simulink model "basebot_turn"  (R2026a)
settings: Solver=VariableStepAuto  MaxStep=1e-4
values from neighbouring files (symbols this model uses):
  B = 0.15    [buildExercise1Models.m]    (also in driveModel.m; driveSquare.m; finalProjectModel.m; squareModel.m = 0.14)
  den = conv([L R], [J D]) + [0 0 K^2]    [compareRobot.m]    (also in driveModel.m; driveSquare.m; piDesign.mat = [3.18211752541e-08 2.39694947115e-05 7.04575028668e-05]; samplingModel.m)
  gear = 9.6    [buildExercise1Models.m]    (also in compareRobot.m; driveModel.m; driveSquare.m; finalProjectModel.m)
  Ki = Kp / 0.04    (= 0.5)    [driveSquare.m]
  Kit = Kpt / 0.15    (= 3.33333333333)    [driveSquare.m]
  Kp = runs{n,2}    [compareRobot.m]    (also in driveSquare.m = 0.02; piDesign.m = 0.13; piDesign.mat = 0.13; samplingModel.m = 0.05)
  Kph = 5    [driveSquare.m]    (also in squareModel.m = 1 / magH(idxWc))
  Kpt = 0.5    [driveSquare.m]
  maxTurn = 5    [driveSquare.m]
  num = K    [compareRobot.m]    (also in driveModel.m; driveSquare.m; piDesign.mat = 0.00812424172394; samplingModel.m)
  r = 0.0315    [compareRobot.m]    (also in driveModel.m; driveSquare.m; finalProjectModel.m; samplingModel.m)
  T = 0.010    (= 0.01)    [compareRobot.m]    (also in piDesign.mat; samplingModel.m; transferFunction.m)
  Ts = 0.001;'    [buildExercise1Models.m]    (also in compareRobot.m = round(median(diff(t)), 4); driveModel.m = 0.001; driveSquare.m = 0.001; finalProjectModel.m = 0.001)
  Vmax = 9    [compareRobot.m]    (also in driveModel.m; driveSquare.m; finalProjectModel.m; piDesign.m = 8)
libraries: slpidlib x3
settings Model: Creator=bidaze  LastModifiedBy=bidaze

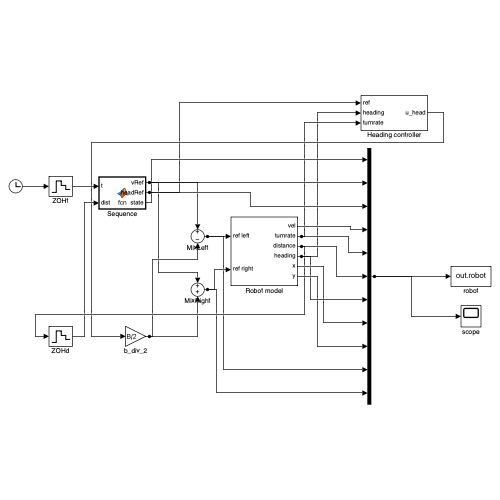
[thumbnail: Simulink's stored preview of the top-level diagram]
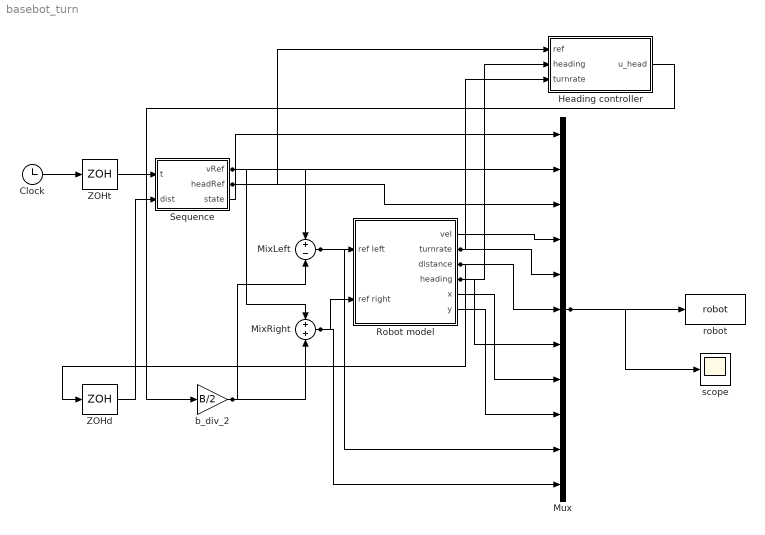
== system basebot_turn ==
  Clock : Clock
  Heading controller : Subsystem
  MixLeft : Sum  Inputs=+-
  MixRight : Sum
  Mux : Mux  Inputs=11
  Robot model : Subsystem
  Sequence : MATLAB Function  TreatAsAtomicUnit=on
  ZOHd : ZeroOrderHold  SampleTime=Ts
  ZOHt : ZeroOrderHold  SampleTime=Ts
  b_div_2 : Gain  Gain=B/2
  robot : ToWorkspace  VariableName=robot  SaveFormat=Timeseries  SampleTime=-1
  scope : Scope
  wires:
  Robot model/5(x) -> Mux/8
  Mux/1 -> scope/1, robot/1
  Robot model/3(distance) -> Mux/6, ZOHd/1
  Robot model/6(y) -> Mux/9
  ZOHt/1 -> Sequence/1(t)
  MixRight/1 -> Robot model/2(ref right), Mux/11
  ZOHd/1 -> Sequence/2(dist)
  Robot model/1(vel) -> Mux/4
  MixLeft/1 -> Robot model/1(ref left), Mux/10
  Robot model/4(heading) -> Mux/7, Heading controller/2(heading)
  Sequence/3(state) -> Mux/1
  Sequence/2(headRef) -> Heading controller/1(ref), Mux/3
  Heading controller/1(u_head) -> b_div_2/1
  Clock/1 -> ZOHt/1
  Robot model/2(turnrate) -> Mux/5, Heading controller/3(turnrate)
  b_div_2/1 -> MixLeft/2, MixRight/2
  Sequence/1(vRef) -> Mux/2, MixLeft/1, MixRight/1

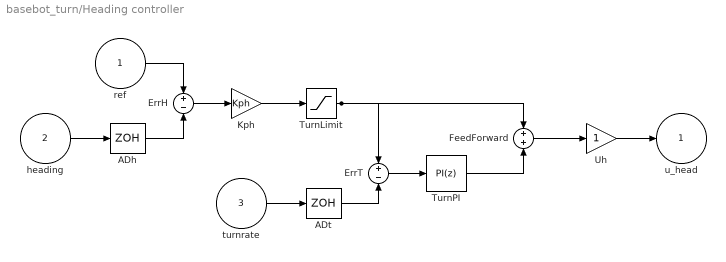
== system basebot_turn/Heading controller ==
  ref : Inport
  heading : Inport  Port=2
  turnrate : Inport  Port=3
  ADh : ZeroOrderHold  SampleTime=Ts
  ADt : ZeroOrderHold  SampleTime=Ts
  ErrH : Sum  Inputs=+-
  ErrT : Sum  Inputs=+-
  FeedForward : Sum
  Kph : Gain  Gain=Kph
  TurnLimit : Saturate  UpperLimit=maxTurn  LowerLimit=-maxTurn
  TurnPI : slpidlib/PID Controller  Controller=PI  Form=Parallel  TimeDomain=Discrete-time  UseExternalTs=off  SampleTime=Ts  IntegratorMethod=Trapezoidal  FilterMethod=Forward Euler  ControllerParametersSource=internal  P=Kpt  I=Kit  UseKiTs=off  D=0  UseExternalDerivativeSource=off  N=100  UseFilter=on  TunerSelectOption=Transfer Function Based (PID Tuner App)  InitialConditionSource=internal  InitialConditionForIntegrator=0  InitialConditionForFilter=0  DifferentiatorICPrevScaledInput=0  ExternalReset=none  TrackingMode=off  Kt=1  LimitOutput=off  SatLimitsSource=internal  UpperSaturationLimit=inf  LowerSaturationLimit=-inf  LinearizeAsGain=off  AntiWindupMode=none  Kb=1  LimitIntegrator=off  UpperIntegratorSaturationLimit=inf  LowerIntegratorSaturationLimit=-inf  POutMin=[]  POutMax=[]  IOutMin=[]  IOutMax=[]  DOutMin=[]  DOutMax=[]  NOutMin=[]  NOutMax=[]  SumOutMin=[]  SumOutMax=[]  SaturationOutMin=[]  SaturationOutMax=[]  PParamMin=[]  PParamMax=[]  IParamMin=[]  IParamMax=[]  DParamMin=[]  DParamMax=[]  NParamMin=[]  NParamMax=[]  KbParamMin=[]  KbParamMax=[]  KtParamMin=[]  KtParamMax=[]  KbOutMin=[]  KbOutMax=[]  KtOutMin=[]  KtOutMax=[]  IntegratorOutMin=[]  IntegratorOutMax=[]  FilterOutMin=[]  FilterOutMax=[]  SumI1OutMin=[]  SumI1OutMax=[]  SumI2OutMin=[]  SumI2OutMax=[]  SumI3OutMin=[]  SumI3OutMax=[]  SumI4OutMin=[]  SumI4OutMax=[]  SumDOutMin=[]  SumDOutMax=[]  DifferentiatorOutMin=[]  DifferentiatorOutMax=[]  FilterDiffOutCoefMin=[]  FilterDiffOutCoefMax=[]  ReciprocalOutMin=[]  ReciprocalOutMax=[]  SumDenOutMin=[]  SumDenOutMax=[]  SumNumOutMin=[]  SumNumOutMax=[]  DivideOutMin=[]  DivideOutMax=[]  UdiffTsProdOutMin=[]  UdiffTsProdOutMax=[]  NTsProdOutMin=[]  NTsProdOutMax=[]  UintegralTsProdOutMin=[]  UintegralTsProdOutMax=[]  UngainTsProdOutMin=[]  UngainTsProdOutMax=[]  ClampingZeroOutDataTypeStr=Inherit: Inherit via back propagation  ClampingZeroOutMin=[]  ClampingZeroOutMax=[]  FilterDenConstantOutDataTypeStr=Inherit: Inherit via back propagation  FilterDenConstantOutMin=[]  FilterDenConstantOutMax=[]  PCopyOutDataTypeStr=Inherit: Inherit via back propagation  PCopyOutMin=[]  PCopyOutMax=[]  NCopyOutDataTypeStr=Inherit: Inherit via back propagation  NCopyOutMin=[]  NCopyOutMax=[]  IntegratorContinuousStateAttributes=''  IntegratorStateMustResolveToSignalObject=off  IntegratorRTWStateStorageClass=Auto  FilterContinuousStateAttributes=''  FilterStateMustResolveToSignalObject=off  FilterRTWStateStorageClass=Auto  ParallelPVariant=InternalParameters  IdealPVariant=Disabled  IVariant=InternalParameters  DVariant=Disabled  IntegratorVariant=Discrete  SatVariant=Disabled  AWVariant=Passthrough  PCopyVariant=Disabled  TRVariant=Disabled  FdbkBlocksVariant=Forward  IdealPFdbkVariant=Disabled  SatFdbkVariant=Disabled  DerivativeFilterVariant=Disabled  NVariant=Disabled  NCopyVariant=Disabled_SignalSpec  FilterICVariant=Disabled  IntegratorICVariant=InternalICs  ExternalResetVariant=Disabled  TRSumVariant=Passthrough  SumFdbkVariant=Disabled  SumVariant=Sum_PI  TsampFilterVariant=InternalTs  TsampNgainVariant=Passthrough  TsampIntegralVariant=Disabled_SignalSpec  ExternalSaturationOutDataTypeStr=Inherit: Same as second input  DerivativeSourceVariant=Disabled  PreIntVariant=InternalPreInt
      settings: LibrarySourceBlock=simulink/Discrete/Discrete PID Controller
  Uh : Gain
  u_head : Outport
  wires:
  Uh/1 -> u_head/1
  FeedForward/1 -> Uh/1
  ADt/1 -> ErrT/2
  TurnLimit/1 -> FeedForward/1, ErrT/1
  ADh/1 -> ErrH/2
  TurnPI/1 -> FeedForward/2
  ErrT/1 -> TurnPI/1
  turnrate/1 -> ADt/1
  Kph/1 -> TurnLimit/1
  ref/1 -> ErrH/1
  ErrH/1 -> Kph/1
  heading/1 -> ADh/1

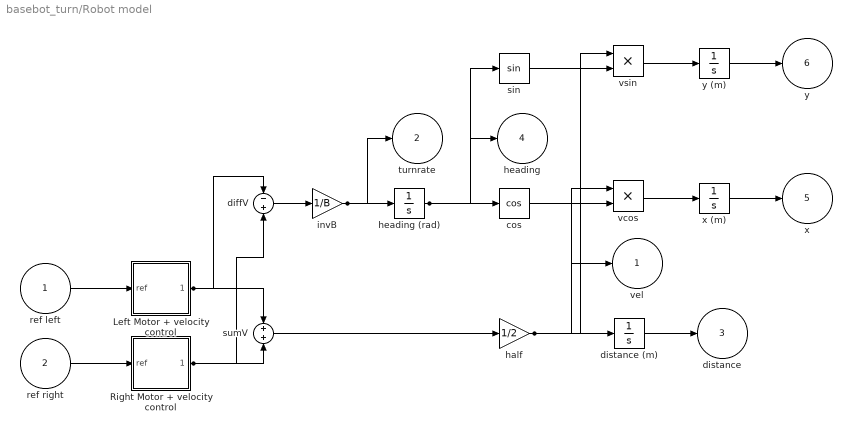
== system basebot_turn/Robot model ==
  ref left : Inport
  ref right : Inport  Port=2
  Left Motor + velocity control : Subsystem
  Right Motor + velocity control : Subsystem
  cos : Trigonometry  Operator=cos
  diffV : Sum  Inputs=-+
  distance (m) : Integrator
  half : Gain  Gain=1/2
  heading (rad) : Integrator
  invB : Gain  Gain=1/B
  sin : Trigonometry
  sumV : Sum
  vcos : Product
  vsin : Product
  x (m) : Integrator
  y (m) : Integrator
  vel : Outport
  turnrate : Outport  Port=2
  distance : Outport  Port=3
  heading : Outport  Port=4
  x : Outport  Port=5
  y : Outport  Port=6
  wires:
  x (m)/1 -> x/1
  y (m)/1 -> y/1
  distance (m)/1 -> distance/1
  vcos/1 -> x (m)/1
  cos/1 -> vcos/2
  heading (rad)/1 -> heading/1, sin/1, cos/1
  Right Motor + velocity control/1(velocity) -> sumV/2, diffV/2
  invB/1 -> turnrate/1, heading (rad)/1
  Left Motor + velocity control/1(velocity) -> diffV/1, sumV/1
  sumV/1 -> half/1
  sin/1 -> vsin/2
  vsin/1 -> y (m)/1
  ref left/1 -> Left Motor + velocity control/1(ref)
  diffV/1 -> invB/1
  half/1 -> vel/1, vcos/1, vsin/1, distance (m)/1
  ref right/1 -> Right Motor + velocity control/1(ref)

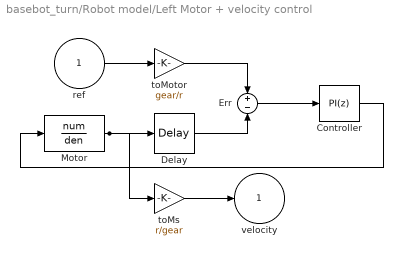
== system basebot_turn/Robot model/Left Motor + velocity control ==
  ref : Inport
  Controller : slpidlib/PID Controller  Controller=PI  Form=Parallel  TimeDomain=Discrete-time  UseExternalTs=off  SampleTime=Ts  IntegratorMethod=Forward Euler  FilterMethod=Forward Euler  ControllerParametersSource=internal  P=Kp  I=Ki  UseKiTs=off  D=0  UseExternalDerivativeSource=off  N=100  UseFilter=on  TunerSelectOption=Transfer Function Based (PID Tuner App)  InitialConditionSource=internal  InitialConditionForIntegrator=0  InitialConditionForFilter=0  DifferentiatorICPrevScaledInput=0  ExternalReset=none  TrackingMode=off  Kt=1  LimitOutput=on  SatLimitsSource=internal  UpperSaturationLimit=Vmax  LowerSaturationLimit=-Vmax  LinearizeAsGain=off  AntiWindupMode=clamping  Kb=1  LimitIntegrator=off  UpperIntegratorSaturationLimit=inf  LowerIntegratorSaturationLimit=-inf  POutMin=[]  POutMax=[]  IOutMin=[]  IOutMax=[]  DOutMin=[]  DOutMax=[]  NOutMin=[]  NOutMax=[]  SumOutMin=[]  SumOutMax=[]  SaturationOutMin=[]  SaturationOutMax=[]  PParamMin=[]  PParamMax=[]  IParamMin=[]  IParamMax=[]  DParamMin=[]  DParamMax=[]  NParamMin=[]  NParamMax=[]  KbParamMin=[]  KbParamMax=[]  KtParamMin=[]  KtParamMax=[]  KbOutMin=[]  KbOutMax=[]  KtOutMin=[]  KtOutMax=[]  IntegratorOutMin=[]  IntegratorOutMax=[]  FilterOutMin=[]  FilterOutMax=[]  SumI1OutMin=[]  SumI1OutMax=[]  SumI2OutMin=[]  SumI2OutMax=[]  SumI3OutMin=[]  SumI3OutMax=[]  SumI4OutMin=[]  SumI4OutMax=[]  SumDOutMin=[]  SumDOutMax=[]  DifferentiatorOutMin=[]  DifferentiatorOutMax=[]  FilterDiffOutCoefMin=[]  FilterDiffOutCoefMax=[]  ReciprocalOutMin=[]  ReciprocalOutMax=[]  SumDenOutMin=[]  SumDenOutMax=[]  SumNumOutMin=[]  SumNumOutMax=[]  DivideOutMin=[]  DivideOutMax=[]  UdiffTsProdOutMin=[]  UdiffTsProdOutMax=[]  NTsProdOutMin=[]  NTsProdOutMax=[]  UintegralTsProdOutMin=[]  UintegralTsProdOutMax=[]  UngainTsProdOutMin=[]  UngainTsProdOutMax=[]  ClampingZeroOutDataTypeStr=Inherit: Inherit via back propagation  ClampingZeroOutMin=[]  ClampingZeroOutMax=[]  FilterDenConstantOutDataTypeStr=Inherit: Inherit via back propagation  FilterDenConstantOutMin=[]  FilterDenConstantOutMax=[]  PCopyOutDataTypeStr=Inherit: Inherit via back propagation  PCopyOutMin=[]  PCopyOutMax=[]  NCopyOutDataTypeStr=Inherit: Inherit via back propagation  NCopyOutMin=[]  NCopyOutMax=[]  IntegratorContinuousStateAttributes=''  IntegratorStateMustResolveToSignalObject=off  IntegratorRTWStateStorageClass=Auto  FilterContinuousStateAttributes=''  FilterStateMustResolveToSignalObject=off  FilterRTWStateStorageClass=Auto  ParallelPVariant=InternalParameters  IdealPVariant=Disabled  IVariant=InternalParameters  DVariant=Disabled  IntegratorVariant=Discrete  SatVariant=Enabled  AWVariant=DiscClampingParallel  PCopyVariant=Disabled  TRVariant=Disabled  FdbkBlocksVariant=Forward  IdealPFdbkVariant=Disabled  SatFdbkVariant=Disabled  DerivativeFilterVariant=Disabled  NVariant=Disabled  NCopyVariant=Disabled_SignalSpec  FilterICVariant=Disabled  IntegratorICVariant=InternalICs  ExternalResetVariant=Disabled  TRSumVariant=Passthrough  SumFdbkVariant=Disabled  SumVariant=Sum_PI  TsampFilterVariant=InternalTs  TsampNgainVariant=Passthrough  TsampIntegralVariant=Disabled_SignalSpec  ExternalSaturationOutDataTypeStr=Inherit: Same as second input  DerivativeSourceVariant=Disabled  PreIntVariant=InternalPreInt
      settings: LibrarySourceBlock=simulink/Discrete/Discrete PID Controller
  Delay : TransportDelay  DelayTime=T
  Err : Sum  Inputs=+-
  Motor : TransferFcn  Numerator=num  Denominator=den
  toMotor : Gain  Gain=gear/r
  toMs : Gain  Gain=r/gear
  velocity : Outport
  wires:
  toMs/1 -> velocity/1
  Delay/1 -> Err/2
  toMotor/1 -> Err/1
  Controller/1 -> Motor/1
  Err/1 -> Controller/1
  Motor/1 -> toMs/1, Delay/1
  ref/1 -> toMotor/1

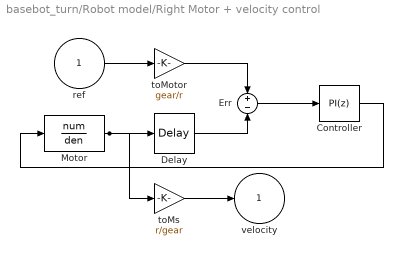
== system basebot_turn/Robot model/Right Motor + velocity control ==
  ref : Inport
  Controller : slpidlib/PID Controller  Controller=PI  Form=Parallel  TimeDomain=Discrete-time  UseExternalTs=off  SampleTime=Ts  IntegratorMethod=Forward Euler  FilterMethod=Forward Euler  ControllerParametersSource=internal  P=Kp  I=Ki  UseKiTs=off  D=0  UseExternalDerivativeSource=off  N=100  UseFilter=on  TunerSelectOption=Transfer Function Based (PID Tuner App)  InitialConditionSource=internal  InitialConditionForIntegrator=0  InitialConditionForFilter=0  DifferentiatorICPrevScaledInput=0  ExternalReset=none  TrackingMode=off  Kt=1  LimitOutput=on  SatLimitsSource=internal  UpperSaturationLimit=Vmax  LowerSaturationLimit=-Vmax  LinearizeAsGain=off  AntiWindupMode=clamping  Kb=1  LimitIntegrator=off  UpperIntegratorSaturationLimit=inf  LowerIntegratorSaturationLimit=-inf  POutMin=[]  POutMax=[]  IOutMin=[]  IOutMax=[]  DOutMin=[]  DOutMax=[]  NOutMin=[]  NOutMax=[]  SumOutMin=[]  SumOutMax=[]  SaturationOutMin=[]  SaturationOutMax=[]  PParamMin=[]  PParamMax=[]  IParamMin=[]  IParamMax=[]  DParamMin=[]  DParamMax=[]  NParamMin=[]  NParamMax=[]  KbParamMin=[]  KbParamMax=[]  KtParamMin=[]  KtParamMax=[]  KbOutMin=[]  KbOutMax=[]  KtOutMin=[]  KtOutMax=[]  IntegratorOutMin=[]  IntegratorOutMax=[]  FilterOutMin=[]  FilterOutMax=[]  SumI1OutMin=[]  SumI1OutMax=[]  SumI2OutMin=[]  SumI2OutMax=[]  SumI3OutMin=[]  SumI3OutMax=[]  SumI4OutMin=[]  SumI4OutMax=[]  SumDOutMin=[]  SumDOutMax=[]  DifferentiatorOutMin=[]  DifferentiatorOutMax=[]  FilterDiffOutCoefMin=[]  FilterDiffOutCoefMax=[]  ReciprocalOutMin=[]  ReciprocalOutMax=[]  SumDenOutMin=[]  SumDenOutMax=[]  SumNumOutMin=[]  SumNumOutMax=[]  DivideOutMin=[]  DivideOutMax=[]  UdiffTsProdOutMin=[]  UdiffTsProdOutMax=[]  NTsProdOutMin=[]  NTsProdOutMax=[]  UintegralTsProdOutMin=[]  UintegralTsProdOutMax=[]  UngainTsProdOutMin=[]  UngainTsProdOutMax=[]  ClampingZeroOutDataTypeStr=Inherit: Inherit via back propagation  ClampingZeroOutMin=[]  ClampingZeroOutMax=[]  FilterDenConstantOutDataTypeStr=Inherit: Inherit via back propagation  FilterDenConstantOutMin=[]  FilterDenConstantOutMax=[]  PCopyOutDataTypeStr=Inherit: Inherit via back propagation  PCopyOutMin=[]  PCopyOutMax=[]  NCopyOutDataTypeStr=Inherit: Inherit via back propagation  NCopyOutMin=[]  NCopyOutMax=[]  IntegratorContinuousStateAttributes=''  IntegratorStateMustResolveToSignalObject=off  IntegratorRTWStateStorageClass=Auto  FilterContinuousStateAttributes=''  FilterStateMustResolveToSignalObject=off  FilterRTWStateStorageClass=Auto  ParallelPVariant=InternalParameters  IdealPVariant=Disabled  IVariant=InternalParameters  DVariant=Disabled  IntegratorVariant=Discrete  SatVariant=Enabled  AWVariant=DiscClampingParallel  PCopyVariant=Disabled  TRVariant=Disabled  FdbkBlocksVariant=Forward  IdealPFdbkVariant=Disabled  SatFdbkVariant=Disabled  DerivativeFilterVariant=Disabled  NVariant=Disabled  NCopyVariant=Disabled_SignalSpec  FilterICVariant=Disabled  IntegratorICVariant=InternalICs  ExternalResetVariant=Disabled  TRSumVariant=Passthrough  SumFdbkVariant=Disabled  SumVariant=Sum_PI  TsampFilterVariant=InternalTs  TsampNgainVariant=Passthrough  TsampIntegralVariant=Disabled_SignalSpec  ExternalSaturationOutDataTypeStr=Inherit: Same as second input  DerivativeSourceVariant=Disabled  PreIntVariant=InternalPreInt
      settings: LibrarySourceBlock=simulink/Discrete/Discrete PID Controller
  Delay : TransportDelay  DelayTime=T
  Err : Sum  Inputs=+-
  Motor : TransferFcn  Numerator=num  Denominator=den
  toMotor : Gain  Gain=gear/r
  toMs : Gain  Gain=r/gear
  velocity : Outport
  wires:
  toMs/1 -> velocity/1
  toMotor/1 -> Err/1
  Controller/1 -> Motor/1
  Motor/1 -> toMs/1, Delay/1
  Err/1 -> Controller/1
  Delay/1 -> Err/2
  ref/1 -> toMotor/1

== matlab function basebot_turn/Sequence ==
  data: t input; vRef output; dist input; headRef output; state output
function [vRef, headRef, state] = fcn(t, dist)
% as SequenceTwoSteps() in basebot_6.ino, MISSION_MODE 2
persistent stopped
if isempty(stopped), stopped = false; end
side = min(4, floor(dist / 0.75));
stopped = stopped || dist >= 5 * 0.75;
headRef = side * pi / 2;
if stopped
    vRef = 0;  state = 2;  headRef = 4 * pi / 2;
elseif t <= 0.1
    vRef = 0;  state = 10;
else
    vRef = 0.75;  state = 11 + side;
end
